simulink model "s_c107m32k_vlbi"  (R2018a)
settings: Solver=VariableStepDiscrete  StartTime=0.0  StopTime=(2^15)*10  RelTol=1e-3
undefined symbols (not defined in the file): fft_stages, n_bits_xengs
libraries: xbsIndex_r4 x23049, casper_library_misc x45, xps_library x4, casper_library_scopes x3, simulink x2
(part 54 of 201)

== system s_c107m32k_vlbi/hmc_ct/hmc_addr_gen ==
  note: Map writes across HMC
      | for performance.
  note: Map the output read to collect like channels.
  note: Read when write switches banks.
  note: Write is linear.
  note: Map writes across HMC
      | for performance.
  sync : Inport
  dv : Inport  Port=2
  d256_0 : Inport  Port=3
  d256_1 : Inport  Port=4
  Concat1 : xbsIndex_r4/Concat  num_inputs=2  dbl_ovrd=off  block_type=concat
  Concat2 : xbsIndex_r4/Concat  num_inputs=2  dbl_ovrd=off  block_type=concat
  Concat3 : xbsIndex_r4/Concat  num_inputs=2  dbl_ovrd=off  block_type=concat
  Concat4 : xbsIndex_r4/Concat  Commented=on  num_inputs=4  dbl_ovrd=off  block_type=concat
  Constant6 : xbsIndex_r4/Constant  const=0  gui_display_data_type=Fixed-point  arith_type=Unsigned  n_bits=27 - (invec_bits + outvec_bits + 1)  bin_pt=0  preci_type=Single  exp_width=8  frac_width=24  explicit_period=on  period=1  equ=P=C  opselect=C  inp2=PCIN>>17  opr=+  inp1=P  carry=CIN  dbl_ovrd=off  block_type=constant
  Constant8 : xbsIndex_r4/Constant  const=0  gui_display_data_type=Fixed-point  arith_type=Unsigned  n_bits=27 - (invec_bits + outvec_bits + 1)  bin_pt=0  preci_type=Single  exp_width=8  frac_width=24  explicit_period=on  period=1  equ=P=C  opselect=C  inp2=PCIN>>17  opr=+  inp1=P  carry=CIN  dbl_ovrd=off  block_type=constant
  Delay{1..2,4,9,12,18..22} (10 alike) : xbsIndex_r4/Delay  rst=off  infoeditControl=Selection of Reset will increase slice count due to use of real FFs and instead of SRLs  en=off  latency=7*3  reg_retiming=on  dbl_ovrd=off  block_type=delay
      settings: infoedit=Hardware notes: A delay line is a chain, each link of which is an SRL16 or SRL32 followed by a flip-flop.
  Delay{5..8,10,30..35} (11 alike) : xbsIndex_r4/Delay  rst=off  infoeditControl=Selection of Reset will increase slice count due to use of real FFs and instead of SRLs  en=off  latency=1  reg_retiming=on  dbl_ovrd=off  block_type=delay
      settings: infoedit=Hardware notes: A delay line is a chain, each link of which is an SRL16 or SRL32 followed by a flip-flop.
  Delay{3,11,13..16,24..29} (12 alike) : xbsIndex_r4/Delay  rst=off  infoeditControl=Selection of Reset will increase slice count due to use of real FFs and instead of SRLs  en=off  latency=3  reg_retiming=on  dbl_ovrd=off  block_type=delay
      settings: infoedit=Hardware notes: A delay line is a chain, each link of which is an SRL16 or SRL32 followed by a flip-flop.
  From : From  Commented=on  GotoTag=sync256
  From163 : From  Commented=on  GotoTag=sync80  TagVisibility=global
  From164 : From  Commented=on  GotoTag=valid80  TagVisibility=global
  From166 : From  Commented=on  GotoTag=ss_arm  TagVisibility=global
  From169 : From  Commented=on  GotoTag=sync80  TagVisibility=global
  From_pfb_d1 : From  Commented=on  GotoTag=time80  TagVisibility=global
  Gateway Out{,1..7} (8 alike) : xbsIndex_r4/Gateway Out  inherit_from_input=off  hdl_port=off  rows=1  columns=1  UseAsDAC=off  DACChannel='1'  interface=None  automatic_assignment=on  address_offset=hex2dec('00')  intf_name=''  intf_description=''  timing_constraint=None  locs_specified=off  LOCs={}  io_standard={}  block_type=gatewayout
  Inverter1 : xbsIndex_r4/Inverter  en=off  latency=0  dbl_ovrd=off  block_type=inv
  Logical6 : xbsIndex_r4/Logical  Commented=on  logical_function=OR  inputs=2  en=off  latency=0  precision=Full  arith_type=Unsigned  n_bits=16  bin_pt=0  align_bp=on  dbl_ovrd=off  block_type=logical
  Register5 : xbsIndex_r4/Register  Commented=on  init=0  rst=on  en=on  dbl_ovrd=off  block_type=register
  Register6 : xbsIndex_r4/Register  Commented=on  init=0  rst=on  en=on  dbl_ovrd=off  block_type=register
  Scope : Scope  NumInputPorts=4
  Scope1 : Scope  NumInputPorts=4
  Slice : xbsIndex_r4/Slice  nbits=16  boolean_output=off  mode=Upper Bit Location + Width  bit1=0  base1=MSB of Input  bit0=0  base0=LSB of Input  dbl_ovrd=off  block_type=slice
  Slice1 : xbsIndex_r4/Slice  nbits=invec_bits+outvec_bits  boolean_output=off  mode=Lower Bit Location + Width  bit1=0  base1=MSB of Input  bit0=0  base0=LSB of Input  dbl_ovrd=off  block_type=slice
  Slice5 : xbsIndex_r4/Slice  nbits=9  boolean_output=off  mode=Lower Bit Location + Width  bit1=0  base1=MSB of Input  bit0=0  base0=LSB of Input  dbl_ovrd=off  block_type=slice
  bank : xbsIndex_r4/Slice  nbits=1  boolean_output=on  mode=Upper Bit Location + Width  bit1=0  base1=MSB of Input  bit0=0  base0=LSB of Input  dbl_ovrd=off  block_type=slice
  bus_expand9 : Subsystem  Commented=on  mask(bus_expand){mode=divisions of equal size, outputNum=4, outputWidth=19, outputBinaryPt=0, outputArithmeticType=0, show_format=off, outputToWorkspace=off, variablePrefix=out, outputToModelAsWell=on}
      mask prompts: outputNum "Number of outputs:"; outputWidth "Output width:"; outputBinaryPt "Output binary point position:"; outputArithmeticType "Output arithmetic type (ufix=0, fix=1, bool=2):"; show_format "Print format string?"; outputToWorkspace "Output to workspace?"; variablePrefix "Variable name prefix:"; outputToModelAsWell "Output to model as well?"
      mask help:
      | Expands a 'bus' made using a bus_create or Xilinx
      | concat block.
      | The input will be divided into the specified number
      | of outputs with the specified arithmetic types.
      | Divisions are made from most significant bit.
      mask init: same as s_c107m32k_vlbi/bus_expand1
      settings: AttributesFormatString=4 outputs
      mask TypeOptions mode: divisions of equal size | divisions of arbitrary size
      mask Callback mode: bus_expand_callback();
      mask Callback outputWidth: bus_expand_callback();
      mask Callback outputToWorkspace: bus_expand_callback();
  edge_detect2 : Subsystem  mask(edge_detect){edge=Rising, polarity=Active High, x_in=[0 0.08 0.08 0.16 0.16 0.24 0.24 0.32 0.32 0.4], y_in=[-1 -1  1  1  1  1  1  1  1  1], x_out=[0.6 0.68 0.68 0.76 0.76 0.84 0.84 0.92 0.92 1], y_out=[-1 -1  1  1 -1 -1 -1 -1 -1 -1]}
      mask prompts: edge "Edge Type"; polarity "Output Polarity"; x_in "Input X Positions"; y_in "Input Y Positions"; x_out "Output X Positions"; y_out "Output Y Positions"
      mask help: Output is active for one-cycle after each edge of the specified type (i.e. rising, falling or both).
      mask init: same as s_c107m32k_vlbi/edge_detect1
      settings: AttributesFormatString=|
      | rising edges
      | active high
      mask Help: Output is active for one-cycle after each edge of the specified type (i.e. rising, falling, or both).  Latency is zero.
      mask TypeOptions edge: Rising | Falling | Both
      mask TypeOptions polarity: Active High | Active Low
      mask Display:
      | plot(x_in_num,0.5+y_in_num*0.2);
      | plot(x_out_num,0.5+y_out_num*0.2);
  edge_detect4 : Subsystem  Commented=on  mask(edge_detect){edge=Rising, polarity=Active High, x_in=[0 0.08 0.08 0.16 0.16 0.24 0.24 0.32 0.32 0.4], y_in=[-1 -1  1  1  1  1  1  1  1  1], x_out=[0.6 0.68 0.68 0.76 0.76 0.84 0.84 0.92 0.92 1], y_out=[-1 -1  1  1 -1 -1 -1 -1 -1 -1]}
      mask prompts: edge "Edge Type"; polarity "Output Polarity"; x_in "Input X Positions"; y_in "Input Y Positions"; x_out "Output X Positions"; y_out "Output Y Positions"
      mask help: Output is active for one-cycle after each edge of the specified type (i.e. rising, falling or both).
      mask init: same as s_c107m32k_vlbi/edge_detect1
      settings: AttributesFormatString=|
      | rising edges
      | active high
      mask Help: Output is active for one-cycle after each edge of the specified type (i.e. rising, falling, or both).  Latency is zero.
      mask TypeOptions edge: Rising | Falling | Both
      mask TypeOptions polarity: Active High | Active Low
      mask Display:
      | plot(x_in_num,0.5+y_in_num*0.2);
      | plot(x_out_num,0.5+y_out_num*0.2);
  edge_detect6 : Subsystem  Commented=on  mask(edge_detect){edge=Rising, polarity=Active High, x_in=[0 0.08 0.08 0.16 0.16 0.24 0.24 0.32 0.32 0.4], y_in=[-1 -1  1  1  1  1  1  1  1  1], x_out=[0.6 0.68 0.68 0.76 0.76 0.84 0.84 0.92 0.92 1], y_out=[-1 -1  1  1 -1 -1 -1 -1 -1 -1]}
      mask prompts: edge "Edge Type"; polarity "Output Polarity"; x_in "Input X Positions"; y_in "Input Y Positions"; x_out "Output X Positions"; y_out "Output Y Positions"
      mask help: Output is active for one-cycle after each edge of the specified type (i.e. rising, falling or both).
      mask init: same as s_c107m32k_vlbi/edge_detect1
      settings: AttributesFormatString=|
      | rising edges
      | active high
      mask Help: Output is active for one-cycle after each edge of the specified type (i.e. rising, falling, or both).  Latency is zero.
      mask TypeOptions edge: Rising | Falling | Both
      mask TypeOptions polarity: Active High | Active Low
      mask Display:
      | plot(x_in_num,0.5+y_in_num*0.2);
      | plot(x_out_num,0.5+y_out_num*0.2);
  hmc_addr_opt : Subsystem
  hmc_addr_opt1 : Subsystem
  last_tag2 : xbsIndex_r4/Register  init=0  rst=on  en=on  dbl_ovrd=off  block_type=register
  rd_add_ctr : Subsystem
  read_map_calc : Subsystem  mask{rmc_invec_bits=invec_bits, rmc_outvec_bits=outvec_bits, lat=3, max_x_boards_bits=max_x_boards_bits, n_bits_chans_per_word=n_bits_chans_per_word, max_x_per_board_bits=max_x_per_board_bits}
      mask prompts: rmc_invec_bits "Input vector bits"; rmc_outvec_bits "output vector bits"; lat "latency per block"; max_x_boards_bits "max x boards (2^?)"; n_bits_chans_per_word "channels per output word (2^?)"; max_x_per_board_bits "max x engines per board (2^?)"
      mask init:
      | display_string = ['latency=', num2str(lat * 7), '\ninput_vector_bits=', num2str(rmc_invec_bits), '\noutput_vector_bits=', num2str(rmc_outvec_bits)];
      | set_param(gcb, 'AttributesFormatString', display_string);
      settings: AttributesFormatString=latency=21\ninput_vector_bits=11\noutput_vector_bits=8
  snap_agen : Subsystem  Tag=casper:bitsnap  Commented=on  AncestorBlock=casper_library_scopes/bitfield_snapshot  mask(bitsnap){io_names=[sync dv time rd_ctr raw_cnt hmc_offset rd_map], io_widths=[1 1 48 19 19 19 19], io_bps=[0 0 0 0 0 0 0], io_types=[2 2 0 0 0 0 0], show_format=on, snap_storage=bram, snap_dram_dimm=2, snap_dram_clock=250, snap_nsamples=12, snap_data_width=128, snap_offset=on, snap_circap=off, snap_value=off, snap_ext_arm=on, snap_ext_circ=off, snap_provide_outputs=on, snap_use_dsp48=on, snap_delay=0, extra_names=[c d], extra_widths=[30 2], extra_bps=[0 0], extra_types=0}
      mask prompts: io_names "Names [msb...lsb]"; io_widths "Bitwidths [msb...lsb]"; io_bps "Binary pts [msb...lsb]"; io_types "Data types [msb...lsb], ufix=0, fix=1, bool=2"; show_format "Print format string?"; snap_storage "Storage medium"; snap_dram_dimm "DRAM dimm"; snap_dram_clock "DRAM clock rate"; snap_nsamples "Number of Samples (2^?)"; snap_data_width "Data width"; snap_offset "Start delay support"; snap_circap "Circular capture support"; snap_value "Extra value capture support"; snap_ext_arm "External arm support"; snap_ext_circ "External circular capture support"; snap_provide_outputs "Provide outputs"; snap_use_dsp48 "Use DSP48s to implement counters"; snap_delay "Pre-snapshot delay"; extra_names "Names [msb...lsb]"; extra_widths "Widths [msb...lsb]"; extra_bps "Binary pts [msb...lsb]"; extra_types "Data types [msb...lsb], ufix=0, fix=1, bool=2"
      mask help:
      | A wrapped snapshot block. Allows specification of inputs to a snapblock word so the toolflow can automatically set up the scope.
      | See documentation for snapshot for explanation of parameters.
      mask init:
      | bitsnap_init(gcb);
      settings: AttributesFormatString=|
      | snap(7):b,b,uf48.0,uf19.0,uf19.0,uf19.0,uf19.0 = 126 bits\n128 wide, 4096 deep
      | debugID: 121595614
      mask TypeOptions snap_storage: bram | dram
      mask Callback snap_storage: bitsnap_callback();
      mask TypeOptions snap_dram_dimm: 1 | 2 | 3 | 4
      mask TypeOptions snap_dram_clock: 200 | 250 | 266 | 300 | 333
      mask TypeOptions snap_data_width: 8 | 16 | 32 | 64 | 128
      mask Callback snap_value: bitsnap_callback();
      mask Callback snap_ext_arm: bitsnap_callback();
      mask Callback snap_ext_circ: bitsnap_callback();
      mask Callback snap_provide_outputs: bitsnap_callback();
      mask DialogControl ParameterTabVar0 Prompt: Inputs
      mask DialogControl ParameterTabVar01 Prompt: Snapshot
      mask DialogControl ParameterTabVar012 Prompt: Extra Value
  spectrum_ctr5 : xbsIndex_r4/Slice  Commented=on  nbits=16  boolean_output=off  mode=Lower Bit Location + Width  bit1=-1  base1=MSB of Input  bit0=32  base0=LSB of Input  dbl_ovrd=off  block_type=slice
  spectrum_ctr6 : xbsIndex_r4/Slice  Commented=on  nbits=32  boolean_output=off  mode=Lower Bit Location + Width  bit1=-1  base1=MSB of Input  bit0=0  base0=LSB of Input  dbl_ovrd=off  block_type=slice
  sync_time_proc_lsw : Subsystem  Tag=xps:sw_reg  Commented=on  AncestorBlock=xps_library/Memory/software_register  mask(swreg){io_dir=To Processor, io_delay=0, init_val=0, sample_period=1, names=lsw, bitwidths=32, bin_pts=0, arith_types=0, sim_port=off, show_format=on}
      mask prompts: io_dir "I/O direction"; io_delay "I/O delay"; init_val "Initial Value"; sample_period "Sample period"; names "Bitfield names [msb...lsb]"; bitwidths "Bitfield widths"; bin_pts "Bitfield binary pts"; arith_types "Bitfield types, ufix=0, fix=1, bool=2"; sim_port "Provide sim input/output?"; show_format "Print format string?"
      mask help: A 32-bit software-accessible register. Can be divided into bitfields of varying widths and types using the fields in the block mask.
      mask init:
      | swreg_init(gcb)
      settings: AttributesFormatString=1output:uf32.0 = 32 bits
      mask TypeOptions io_dir: To Processor | From Processor
      mask Callback io_dir:
      | mask_enables = get_param(gcb, 'MaskEnables');
      | mask_names = get_param(gcb, 'MaskNames');
      | if strcmp(get_param(gcb, 'io_dir'), 'To Processor'),
      |     mask_enables{ismember(mask_names, 'sample_period')} = 'off';
      | else
      |     mask_enables{ismember(mask_names, 'sample_period')} = 'on';
      | end
      | set_param(gcb, 'MaskEnables', mask_enables);
      mask DialogControl ParameterTabVar0 Prompt: Setup
  sync_time_proc_msw : Subsystem  Tag=xps:sw_reg  Commented=on  AncestorBlock=xps_library/Memory/software_register  mask(swreg){io_dir=To Processor, io_delay=0, init_val=0, sample_period=1, names=msw, bitwidths=16, bin_pts=0, arith_types=0, sim_port=off, show_format=on}
      mask prompts: io_dir "I/O direction"; io_delay "I/O delay"; init_val "Initial Value"; sample_period "Sample period"; names "Bitfield names [msb...lsb]"; bitwidths "Bitfield widths"; bin_pts "Bitfield binary pts"; arith_types "Bitfield types, ufix=0, fix=1, bool=2"; sim_port "Provide sim input/output?"; show_format "Print format string?"
      mask help: A 32-bit software-accessible register. Can be divided into bitfields of varying widths and types using the fields in the block mask.
      mask init:
      | swreg_init(gcb)
      settings: AttributesFormatString=1output:uf16.0 = 16 bits
      mask TypeOptions io_dir: To Processor | From Processor
      mask Callback io_dir:
      | mask_enables = get_param(gcb, 'MaskEnables');
      | mask_names = get_param(gcb, 'MaskNames');
      | if strcmp(get_param(gcb, 'io_dir'), 'To Processor'),
      |     mask_enables{ismember(mask_names, 'sample_period')} = 'off';
      | else
      |     mask_enables{ismember(mask_names, 'sample_period')} = 'on';
      | end
      | set_param(gcb, 'MaskEnables', mask_enables);
      mask DialogControl ParameterTabVar0 Prompt: Setup
  time_gen_1 : Subsystem  Commented=on  mask{n_bits_period=0, n_bits_increment=3, n_bits_counter=48}
      mask prompts: n_bits_period "Period (2^?)"; n_bits_increment "Increment (2^?)"; n_bits_counter "Counter size (2^?)"
  waddr : xbsIndex_r4/Counter  cnt_type=Free Running  cnt_to=Inf  operation=Up  start_count=0  cnt_by_val=1  arith_type=Unsigned  n_bits=invec_bits + outvec_bits + 1  bin_pt=0  load_pin=off  rst=on  en=on  explicit_period=on  period=1  use_behavioral_HDL=off  implementation=Fabric  dbl_ovrd=off  block_type=counter
  we_delay1 : Subsystem  Tag=cmac_delinked  Commented=on  mask(pipeline){csp_latency=2}
      mask prompts: csp_latency "Latency"
      mask help:
      | An explicitly laid-out delay line to avoid mapping to SRL16s
      | for use in pipelining to help achieve timing closure.
      mask init:
      | pipeline_init(gcb,'latency',csp_latency);
      settings: AttributesFormatString=Latency = %<latency>
      mask Display:
      | port_label('input', 1, 'd');
      | port_label('output', 1, 'q');
      | disp(['Z^-', num2str(csp_latency)]);
  we_delay10 : Subsystem  Tag=cmac_delinked  Commented=on  mask(pipeline){csp_latency=2}
      mask prompts: csp_latency "Latency"
      mask help:
      | An explicitly laid-out delay line to avoid mapping to SRL16s
      | for use in pipelining to help achieve timing closure.
      mask init:
      | pipeline_init(gcb,'latency',csp_latency);
      settings: AttributesFormatString=Latency = %<latency>
      mask Display:
      | port_label('input', 1, 'd');
      | port_label('output', 1, 'q');
      | disp(['Z^-', num2str(csp_latency)]);
  we_delay12 : Subsystem  Tag=cmac_delinked  Commented=on  mask(pipeline){csp_latency=2}
      mask prompts: csp_latency "Latency"
      mask help:
      | An explicitly laid-out delay line to avoid mapping to SRL16s
      | for use in pipelining to help achieve timing closure.
      mask init:
      | pipeline_init(gcb,'latency',csp_latency);
      settings: AttributesFormatString=Latency = %<latency>
      mask Display:
      | port_label('input', 1, 'd');
      | port_label('output', 1, 'q');
      | disp(['Z^-', num2str(csp_latency)]);
  we_delay13 : Subsystem  Tag=cmac_delinked  Commented=on  mask(pipeline){csp_latency=2}
      mask prompts: csp_latency "Latency"
      mask help:
      | An explicitly laid-out delay line to avoid mapping to SRL16s
      | for use in pipelining to help achieve timing closure.
      mask init:
      | pipeline_init(gcb,'latency',csp_latency);
      settings: AttributesFormatString=Latency = %<latency>
      mask Display:
      | port_label('input', 1, 'd');
      | port_label('output', 1, 'q');
      | disp(['Z^-', num2str(csp_latency)]);
  we_delay2 : Subsystem  Tag=cmac_delinked  Commented=on  mask(pipeline){csp_latency=2}
      mask prompts: csp_latency "Latency"
      mask help:
      | An explicitly laid-out delay line to avoid mapping to SRL16s
      | for use in pipelining to help achieve timing closure.
      mask init:
      | pipeline_init(gcb,'latency',csp_latency);
      settings: AttributesFormatString=Latency = %<latency>
      mask Display:
      | port_label('input', 1, 'd');
      | port_label('output', 1, 'q');
      | disp(['Z^-', num2str(csp_latency)]);
  we_delay3 : Subsystem  Tag=cmac_delinked  Commented=on  mask(pipeline){csp_latency=2}
      mask prompts: csp_latency "Latency"
      mask help:
      | An explicitly laid-out delay line to avoid mapping to SRL16s
      | for use in pipelining to help achieve timing closure.
      mask init:
      | pipeline_init(gcb,'latency',csp_latency);
      settings: AttributesFormatString=Latency = %<latency>
      mask Display:
      | port_label('input', 1, 'd');
      | port_label('output', 1, 'q');
      | disp(['Z^-', num2str(csp_latency)]);
  we_delay4 : Subsystem  Tag=cmac_delinked  Commented=on  mask(pipeline){csp_latency=2}
      mask prompts: csp_latency "Latency"
      mask help:
      | An explicitly laid-out delay line to avoid mapping to SRL16s
      | for use in pipelining to help achieve timing closure.
      mask init:
      | pipeline_init(gcb,'latency',csp_latency);
      settings: AttributesFormatString=Latency = %<latency>
      mask Display:
      | port_label('input', 1, 'd');
      | port_label('output', 1, 'q');
      | disp(['Z^-', num2str(csp_latency)]);
  we_delay6 : Subsystem  Tag=cmac_delinked  Commented=on  mask(pipeline){csp_latency=2}
      mask prompts: csp_latency "Latency"
      mask help:
      | An explicitly laid-out delay line to avoid mapping to SRL16s
      | for use in pipelining to help achieve timing closure.
      mask init:
      | pipeline_init(gcb,'latency',csp_latency);
      settings: AttributesFormatString=Latency = %<latency>
      mask Display:
      | port_label('input', 1, 'd');
      | port_label('output', 1, 'q');
      | disp(['Z^-', num2str(csp_latency)]);
  we_delay8 : Subsystem  Tag=cmac_delinked  Commented=on  mask(pipeline){csp_latency=2}
      mask prompts: csp_latency "Latency"
      mask help:
      | An explicitly laid-out delay line to avoid mapping to SRL16s
      | for use in pipelining to help achieve timing closure.
      mask init:
      | pipeline_init(gcb,'latency',csp_latency);
      settings: AttributesFormatString=Latency = %<latency>
      mask Display:
      | port_label('input', 1, 'd');
      | port_label('output', 1, 'q');
      | disp(['Z^-', num2str(csp_latency)]);
  we_delay9 : Subsystem  Tag=cmac_delinked  Commented=on  mask(pipeline){csp_latency=2}
      mask prompts: csp_latency "Latency"
      mask help:
      | An explicitly laid-out delay line to avoid mapping to SRL16s
      | for use in pipelining to help achieve timing closure.
      mask init:
      | pipeline_init(gcb,'latency',csp_latency);
      settings: AttributesFormatString=Latency = %<latency>
      mask Display:
      | port_label('input', 1, 'd');
      | port_label('output', 1, 'q');
      | disp(['Z^-', num2str(csp_latency)]);
  wr_sync : Outport
  wr_en : Outport  Port=2
  wr_addr : Outport  Port=3
  wr_d256_0 : Outport  Port=4
  wr_d256_1 : Outport  Port=5
  rd_en : Outport  Port=6
  rd_addr : Outport  Port=7
  rd_tag : Outport  Port=8
  rd_addr_arm : Outport  Port=9
  rd_arm_raw : Outport  Port=10
  wires:
  Delay14/1 -> Delay21/1
  Inverter1/1 -> Delay8/1  "IN_bank"
  Delay9/1 -> Gateway Out1/1, [wr_dv]
  Delay18/1 -> Slice/1, [wr_d256_0]
  Delay19/1 -> Gateway Out4/1, [wr_sync]
  Delay16/1 -> Delay2/1  "ZEN_en_input"
  Delay25/1 -> Delay9/1  "ZEN_wr_dv"
  Delay27/1 -> Delay18/1
  Delay28/1 -> Delay19/1
  d256_0/1 -> Delay32/1
  Delay11/1 -> Delay4/1
  Delay29/1 -> Delay20/1
  Concat1/1 -> [rd_addr]
  Delay4/1 -> [rd_addr_arm]  "zen_addr_arm"
  Delay2/1 -> [rd_en], Gateway Out5/1  "zen_rden"
  [rd_now] -> last_tag2/3, last_tag2/1
  Delay1/1 -> [rd_tag]  "zen_rdtag"
  dv/1 -> Delay30/1, time_gen_1/5(rd_en), rd_add_ctr/2(dv), Delay6/1, waddr/2  "IN_dv"
  waddr/1 -> [wr_addr_cnt], Delay34/1, Slice5/1, Slice1/1, bank/1  "waddr_cnt"
  sync/1 -> Delay35/1, [sync256], waddr/1, rd_add_ctr/1(rd_now), Delay33/1  "IN_sync"
  Delay20/1 -> Gateway Out2/1, hmc_addr_opt/1(addr)  "ZEN_wrctr"
  hmc_addr_opt/1(" addr_opt") -> Concat2/2
  Concat2/1 -> [wr_addr]
  Constant6/1 -> Concat1/1
  Constant8/1 -> Concat2/1
  Delay34/1 -> Delay29/1
  Delay33/1 -> Delay28/1
  Delay32/1 -> Delay27/1
  Delay30/1 -> Delay25/1
  last_tag2/1 -> Delay10/1, [rd_addr_arm_raw]
  [wr_addr] -> wr_addr/1
  [wr_d256_0] -> wr_d256_0/1
  [rd_en] -> rd_en/1
  [rd_addr] -> rd_addr/1
  [rd_tag] -> rd_tag/1
  [wr_sync] -> wr_sync/1
  [rd_addr_arm] -> rd_addr_arm/1
  [rd_addr_arm_raw] -> rd_arm_raw/1
  [wr_dv] -> wr_en/1
  hmc_addr_opt1/1(" addr_opt") -> Concat1/2
  read_map_calc/1(address) -> Concat4/4, Concat3/2, Gateway Out6/1  "zen_calc_addr"
  Delay21/1 -> Concat3/1  "zen_bank"
  Delay15/1 -> Delay1/1
  rd_add_ctr/1(rd_ctr) -> Delay13/1
  [ct_board_hmc_offset] -> Concat4/3, rd_add_ctr/3(xeng_offset)
  Delay6/1 -> Delay16/1
  Delay8/1 -> Delay14/1
  Delay7/1 -> Delay15/1
  Delay10/1 -> Delay11/1
  Delay13/1 -> Concat4/1, read_map_calc/1(raw_address)
  Slice5/1 -> Delay7/1
  [sync256] -> last_tag2/2
  d256_1/1 -> Delay31/1
  Delay26/1 -> Delay12/1
  Delay31/1 -> Delay26/1
  Delay12/1 -> [wr_d256_1]
  [wr_d256_1] -> wr_d256_1/1
  Gateway Out/1 -> Scope/1
  Delay35/1 -> Delay24/1
  Delay24/1 -> Delay22/1
  Gateway Out1/1 -> Scope/2
  Gateway Out2/1 -> Scope/3
  Slice/1 -> Gateway Out3/1
  Gateway Out3/1 -> Scope/4
  Concat3/1 -> Gateway Out7/1, hmc_addr_opt1/1(addr)  "ZEN_wrctr"
  Gateway Out4/1 -> Scope1/1
  Delay22/1 -> Gateway Out/1
  Gateway Out5/1 -> Scope1/2
  Gateway Out6/1 -> Scope1/3
  Gateway Out7/1 -> Scope1/4
  Slice1/1 -> Delay5/1
  bank/1 -> edge_detect2/1(in), Inverter1/1  "wrbank"
  edge_detect2/1(out) -> [rd_now]
  Delay3/1 -> Concat4/2, read_map_calc/2(raw_cnt)
  Delay5/1 -> Delay3/1
  spectrum_ctr5/1 -> Register6/1
  we_delay10/1(q) -> snap_agen/8(we)
  we_delay2/1(q) -> snap_agen/1(in_sync)
  From_pfb_d1/1 -> time_gen_1/3(wr_val_in)
  time_gen_1/1(rd_sync_out) -> edge_detect6/1(in), we_delay2/1(d), edge_detect4/1(in), Logical6/2
  From163/1 -> time_gen_1/1(wr_sync_in)
  Logical6/1 -> we_delay10/1(d)
  time_gen_1/2(rd_dvalid) -> Logical6/1, we_delay6/1(d)
  From169/1 -> Register5/2, Register6/2
  From166/1 -> snap_agen/10(arm)
  edge_detect4/1(out) -> snap_agen/9(trig)
  we_delay13/1(q) -> sync_time_proc_lsw/1(out_lsw)
  we_delay6/1(q) -> snap_agen/2(in_dv)
  edge_detect6/1(out) -> Register5/3, Register6/3
  From164/1 -> time_gen_1/2(wr_en)
  Register6/1 -> we_delay12/1(d)
  time_gen_1/3(rd_val_out) -> spectrum_ctr5/1, spectrum_ctr6/1, we_delay8/1(d)
  we_delay12/1(q) -> sync_time_proc_msw/1(out_msw)
  From/1 -> time_gen_1/4(rd_sync_in)
  spectrum_ctr6/1 -> Register5/1
  Register5/1 -> we_delay13/1(d)
  we_delay8/1(q) -> snap_agen/3(in_time)
  Concat4/1 -> time_gen_1/6(rd_misc_in)
  we_delay9/1(q) -> snap_agen/7(in_rd_map)
  we_delay1/1(q) -> snap_agen/6(in_hmc_offset)
  we_delay3/1(q) -> snap_agen/5(in_raw_cnt)
  we_delay4/1(q) -> snap_agen/4(in_rd_ctr)
  bus_expand9/1(msb_out4) -> we_delay4/1(d)
  bus_expand9/2(out3) -> we_delay3/1(d)
  bus_expand9/4(lsb_out1) -> we_delay9/1(d)
  bus_expand9/3(out2) -> we_delay1/1(d)
  time_gen_1/4(rd_misc_out) -> bus_expand9/1(bus_in)

== system s_c107m32k_vlbi/hmc_ct/match ==
  dv : Inport
  data : Inport  Port=2
  match_value : Inport  Port=3
  Delay1 : xbsIndex_r4/Delay  rst=off  infoeditControl=Selection of Reset will increase slice count due to use of real FFs and instead of SRLs  en=off  latency=1  reg_retiming=off  dbl_ovrd=off  block_type=delay
  Logical : xbsIndex_r4/Logical  logical_function=AND  inputs=2  en=off  latency=1  precision=Full  arith_type=Unsigned  n_bits=16  bin_pt=0  align_bp=on  dbl_ovrd=off  block_type=logical
  Relational5 : xbsIndex_r4/Relational  mode=a=b  op_type=Bool  en=off  latency=1  dbl_ovrd=off  block_type=relational
      settings: SourceProductName=The database /home/jmanley/.matlab/R2018a/slblocks_master.db is locked, or a table in the database is locked. (database is locked)
  Out1 : Outport
  wires:
  dv/1 -> Delay1/1
  data/1 -> Relational5/1
  match_value/1 -> Relational5/2
  Relational5/1 -> Logical/1
  Delay1/1 -> Logical/2
  Logical/1 -> Out1/1
